simulink subsystem "Controller_v2"  (R2025b)
settings: Solver=VariableStepAuto  StartTime=0.0  StopTime=10.0  RelTol=1e-3
libraries: slpidlib x12
(part 2 of 2)

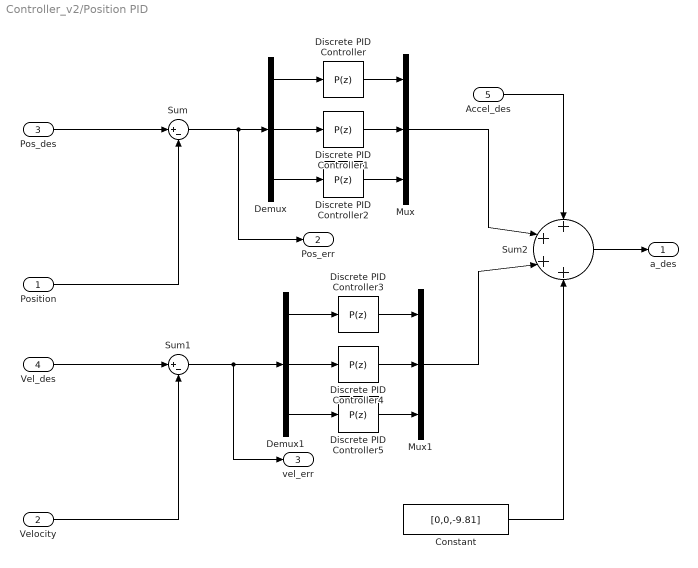
== system Controller_v2/Position PID ==
  Position : Inport
  Velocity : Inport  Port=2
  Pos_des : Inport  Port=3
  Vel_des : Inport  Port=4
  Accel_des : Inport  Port=5
  Constant : Constant  Value=[0,0,-9.81]
  Demux : Demux  Outputs=3
  Demux1 : Demux  Outputs=3
  Discrete PID Controller : slpidlib/PID Controller  Controller=P  Form=Parallel  TimeDomain=Discrete-time  UseExternalTs=off  SampleTime=1/120  IntegratorMethod=Forward Euler  FilterMethod=Forward Euler  ControllerParametersSource=internal  P=0.3  I=0  UseKiTs=off  D=0  UseExternalDerivativeSource=off  N=100  UseFilter=on  TunerSelectOption=Transfer Function Based (PID Tuner App)  InitialConditionSource=internal  InitialConditionForIntegrator=0  InitialConditionForFilter=0  DifferentiatorICPrevScaledInput=0  ExternalReset=none  TrackingMode=off  Kt=1  LimitOutput=off  SatLimitsSource=internal  UpperSaturationLimit=inf  LowerSaturationLimit=-inf  LinearizeAsGain=off  AntiWindupMode=none  Kb=1  LimitIntegrator=off  UpperIntegratorSaturationLimit=inf  LowerIntegratorSaturationLimit=-inf  POutMin=[]  POutMax=[]  IOutMin=[]  IOutMax=[]  DOutMin=[]  DOutMax=[]  NOutMin=[]  NOutMax=[]  SumOutMin=[]  SumOutMax=[]  SaturationOutMin=[]  SaturationOutMax=[]  PParamMin=[]  PParamMax=[]  IParamMin=[]  IParamMax=[]  DParamMin=[]  DParamMax=[]  NParamMin=[]  NParamMax=[]  KbParamMin=[]  KbParamMax=[]  KtParamMin=[]  KtParamMax=[]  KbOutMin=[]  KbOutMax=[]  KtOutMin=[]  KtOutMax=[]  IntegratorOutMin=[]  IntegratorOutMax=[]  FilterOutMin=[]  FilterOutMax=[]  SumI1OutMin=[]  SumI1OutMax=[]  SumI2OutMin=[]  SumI2OutMax=[]  SumI3OutMin=[]  SumI3OutMax=[]  SumI4OutMin=[]  SumI4OutMax=[]  SumDOutMin=[]  SumDOutMax=[]  DifferentiatorOutMin=[]  DifferentiatorOutMax=[]  FilterDiffOutCoefMin=[]  FilterDiffOutCoefMax=[]  ReciprocalOutMin=[]  ReciprocalOutMax=[]  SumDenOutMin=[]  SumDenOutMax=[]  SumNumOutMin=[]  SumNumOutMax=[]  DivideOutMin=[]  DivideOutMax=[]  UdiffTsProdOutMin=[]  UdiffTsProdOutMax=[]  NTsProdOutMin=[]  NTsProdOutMax=[]  UintegralTsProdOutMin=[]  UintegralTsProdOutMax=[]  UngainTsProdOutMin=[]  UngainTsProdOutMax=[]  ClampingZeroOutDataTypeStr=Inherit: Inherit via back propagation  ClampingZeroOutMin=[]  ClampingZeroOutMax=[]  FilterDenConstantOutDataTypeStr=Inherit: Inherit via back propagation  FilterDenConstantOutMin=[]  FilterDenConstantOutMax=[]  PCopyOutDataTypeStr=Inherit: Inherit via back propagation  PCopyOutMin=[]  PCopyOutMax=[]  NCopyOutDataTypeStr=Inherit: Inherit via back propagation  NCopyOutMin=[]  NCopyOutMax=[]  IntegratorContinuousStateAttributes=''  IntegratorStateMustResolveToSignalObject=off  IntegratorRTWStateStorageClass=Auto  FilterContinuousStateAttributes=''  FilterStateMustResolveToSignalObject=off  FilterRTWStateStorageClass=Auto  ParallelPVariant=InternalParameters  IdealPVariant=Disabled  IVariant=Disabled  DVariant=Disabled  IntegratorVariant=Disabled  SatVariant=Disabled  AWVariant=Disabled  PCopyVariant=Disabled  TRVariant=Disabled  FdbkBlocksVariant=Forward  IdealPFdbkVariant=Disabled  SatFdbkVariant=Disabled  DerivativeFilterVariant=Disabled  NVariant=Disabled  NCopyVariant=Disabled_SignalSpec  FilterICVariant=Disabled  IntegratorICVariant=Disabled  ExternalResetVariant=Disabled  TRSumVariant=Passthrough  SumFdbkVariant=Disabled  SumVariant=Passthrough_P  TsampFilterVariant=InternalTs  TsampNgainVariant=Passthrough  TsampIntegralVariant=Disabled_SignalSpec  ExternalSaturationOutDataTypeStr=Inherit: Same as second input  DerivativeSourceVariant=Disabled  PreIntVariant=InternalPreInt
      settings: LibrarySourceBlock=simulink/Discrete/Discrete PID Controller
  Discrete PID Controller1 : slpidlib/PID Controller  Controller=P  Form=Parallel  TimeDomain=Discrete-time  UseExternalTs=off  SampleTime=1/120  IntegratorMethod=Forward Euler  FilterMethod=Forward Euler  ControllerParametersSource=internal  P=0.3  I=0  UseKiTs=off  D=0  UseExternalDerivativeSource=off  N=100  UseFilter=on  TunerSelectOption=Transfer Function Based (PID Tuner App)  InitialConditionSource=internal  InitialConditionForIntegrator=0  InitialConditionForFilter=0  DifferentiatorICPrevScaledInput=0  ExternalReset=none  TrackingMode=off  Kt=1  LimitOutput=off  SatLimitsSource=internal  UpperSaturationLimit=inf  LowerSaturationLimit=-inf  LinearizeAsGain=off  AntiWindupMode=none  Kb=1  LimitIntegrator=off  UpperIntegratorSaturationLimit=inf  LowerIntegratorSaturationLimit=-inf  POutMin=[]  POutMax=[]  IOutMin=[]  IOutMax=[]  DOutMin=[]  DOutMax=[]  NOutMin=[]  NOutMax=[]  SumOutMin=[]  SumOutMax=[]  SaturationOutMin=[]  SaturationOutMax=[]  PParamMin=[]  PParamMax=[]  IParamMin=[]  IParamMax=[]  DParamMin=[]  DParamMax=[]  NParamMin=[]  NParamMax=[]  KbParamMin=[]  KbParamMax=[]  KtParamMin=[]  KtParamMax=[]  KbOutMin=[]  KbOutMax=[]  KtOutMin=[]  KtOutMax=[]  IntegratorOutMin=[]  IntegratorOutMax=[]  FilterOutMin=[]  FilterOutMax=[]  SumI1OutMin=[]  SumI1OutMax=[]  SumI2OutMin=[]  SumI2OutMax=[]  SumI3OutMin=[]  SumI3OutMax=[]  SumI4OutMin=[]  SumI4OutMax=[]  SumDOutMin=[]  SumDOutMax=[]  DifferentiatorOutMin=[]  DifferentiatorOutMax=[]  FilterDiffOutCoefMin=[]  FilterDiffOutCoefMax=[]  ReciprocalOutMin=[]  ReciprocalOutMax=[]  SumDenOutMin=[]  SumDenOutMax=[]  SumNumOutMin=[]  SumNumOutMax=[]  DivideOutMin=[]  DivideOutMax=[]  UdiffTsProdOutMin=[]  UdiffTsProdOutMax=[]  NTsProdOutMin=[]  NTsProdOutMax=[]  UintegralTsProdOutMin=[]  UintegralTsProdOutMax=[]  UngainTsProdOutMin=[]  UngainTsProdOutMax=[]  ClampingZeroOutDataTypeStr=Inherit: Inherit via back propagation  ClampingZeroOutMin=[]  ClampingZeroOutMax=[]  FilterDenConstantOutDataTypeStr=Inherit: Inherit via back propagation  FilterDenConstantOutMin=[]  FilterDenConstantOutMax=[]  PCopyOutDataTypeStr=Inherit: Inherit via back propagation  PCopyOutMin=[]  PCopyOutMax=[]  NCopyOutDataTypeStr=Inherit: Inherit via back propagation  NCopyOutMin=[]  NCopyOutMax=[]  IntegratorContinuousStateAttributes=''  IntegratorStateMustResolveToSignalObject=off  IntegratorRTWStateStorageClass=Auto  FilterContinuousStateAttributes=''  FilterStateMustResolveToSignalObject=off  FilterRTWStateStorageClass=Auto  ParallelPVariant=InternalParameters  IdealPVariant=Disabled  IVariant=Disabled  DVariant=Disabled  IntegratorVariant=Disabled  SatVariant=Disabled  AWVariant=Disabled  PCopyVariant=Disabled  TRVariant=Disabled  FdbkBlocksVariant=Forward  IdealPFdbkVariant=Disabled  SatFdbkVariant=Disabled  DerivativeFilterVariant=Disabled  NVariant=Disabled  NCopyVariant=Disabled_SignalSpec  FilterICVariant=Disabled  IntegratorICVariant=Disabled  ExternalResetVariant=Disabled  TRSumVariant=Passthrough  SumFdbkVariant=Disabled  SumVariant=Passthrough_P  TsampFilterVariant=InternalTs  TsampNgainVariant=Passthrough  TsampIntegralVariant=Disabled_SignalSpec  ExternalSaturationOutDataTypeStr=Inherit: Same as second input  DerivativeSourceVariant=Disabled  PreIntVariant=InternalPreInt
      settings: LibrarySourceBlock=simulink/Discrete/Discrete PID Controller
  Discrete PID Controller2 : slpidlib/PID Controller  Controller=P  Form=Parallel  TimeDomain=Discrete-time  UseExternalTs=off  SampleTime=1/120  IntegratorMethod=Forward Euler  FilterMethod=Forward Euler  ControllerParametersSource=internal  P=2.5  I=0  UseKiTs=off  D=0  UseExternalDerivativeSource=off  N=100  UseFilter=on  TunerSelectOption=Transfer Function Based (PID Tuner App)  InitialConditionSource=internal  InitialConditionForIntegrator=0  InitialConditionForFilter=0  DifferentiatorICPrevScaledInput=0  ExternalReset=none  TrackingMode=off  Kt=1  LimitOutput=off  SatLimitsSource=internal  UpperSaturationLimit=inf  LowerSaturationLimit=-inf  LinearizeAsGain=off  AntiWindupMode=none  Kb=1  LimitIntegrator=off  UpperIntegratorSaturationLimit=inf  LowerIntegratorSaturationLimit=-inf  POutMin=[]  POutMax=[]  IOutMin=[]  IOutMax=[]  DOutMin=[]  DOutMax=[]  NOutMin=[]  NOutMax=[]  SumOutMin=[]  SumOutMax=[]  SaturationOutMin=[]  SaturationOutMax=[]  PParamMin=[]  PParamMax=[]  IParamMin=[]  IParamMax=[]  DParamMin=[]  DParamMax=[]  NParamMin=[]  NParamMax=[]  KbParamMin=[]  KbParamMax=[]  KtParamMin=[]  KtParamMax=[]  KbOutMin=[]  KbOutMax=[]  KtOutMin=[]  KtOutMax=[]  IntegratorOutMin=[]  IntegratorOutMax=[]  FilterOutMin=[]  FilterOutMax=[]  SumI1OutMin=[]  SumI1OutMax=[]  SumI2OutMin=[]  SumI2OutMax=[]  SumI3OutMin=[]  SumI3OutMax=[]  SumI4OutMin=[]  SumI4OutMax=[]  SumDOutMin=[]  SumDOutMax=[]  DifferentiatorOutMin=[]  DifferentiatorOutMax=[]  FilterDiffOutCoefMin=[]  FilterDiffOutCoefMax=[]  ReciprocalOutMin=[]  ReciprocalOutMax=[]  SumDenOutMin=[]  SumDenOutMax=[]  SumNumOutMin=[]  SumNumOutMax=[]  DivideOutMin=[]  DivideOutMax=[]  UdiffTsProdOutMin=[]  UdiffTsProdOutMax=[]  NTsProdOutMin=[]  NTsProdOutMax=[]  UintegralTsProdOutMin=[]  UintegralTsProdOutMax=[]  UngainTsProdOutMin=[]  UngainTsProdOutMax=[]  ClampingZeroOutDataTypeStr=Inherit: Inherit via back propagation  ClampingZeroOutMin=[]  ClampingZeroOutMax=[]  FilterDenConstantOutDataTypeStr=Inherit: Inherit via back propagation  FilterDenConstantOutMin=[]  FilterDenConstantOutMax=[]  PCopyOutDataTypeStr=Inherit: Inherit via back propagation  PCopyOutMin=[]  PCopyOutMax=[]  NCopyOutDataTypeStr=Inherit: Inherit via back propagation  NCopyOutMin=[]  NCopyOutMax=[]  IntegratorContinuousStateAttributes=''  IntegratorStateMustResolveToSignalObject=off  IntegratorRTWStateStorageClass=Auto  FilterContinuousStateAttributes=''  FilterStateMustResolveToSignalObject=off  FilterRTWStateStorageClass=Auto  ParallelPVariant=InternalParameters  IdealPVariant=Disabled  IVariant=Disabled  DVariant=Disabled  IntegratorVariant=Disabled  SatVariant=Disabled  AWVariant=Disabled  PCopyVariant=Disabled  TRVariant=Disabled  FdbkBlocksVariant=Forward  IdealPFdbkVariant=Disabled  SatFdbkVariant=Disabled  DerivativeFilterVariant=Disabled  NVariant=Disabled  NCopyVariant=Disabled_SignalSpec  FilterICVariant=Disabled  IntegratorICVariant=Disabled  ExternalResetVariant=Disabled  TRSumVariant=Passthrough  SumFdbkVariant=Disabled  SumVariant=Passthrough_P  TsampFilterVariant=InternalTs  TsampNgainVariant=Passthrough  TsampIntegralVariant=Disabled_SignalSpec  ExternalSaturationOutDataTypeStr=Inherit: Same as second input  DerivativeSourceVariant=Disabled  PreIntVariant=InternalPreInt
      settings: LibrarySourceBlock=simulink/Discrete/Discrete PID Controller
  Discrete PID Controller3 : slpidlib/PID Controller  Controller=P  Form=Parallel  TimeDomain=Discrete-time  UseExternalTs=off  SampleTime=1/120  IntegratorMethod=Forward Euler  FilterMethod=Forward Euler  ControllerParametersSource=internal  P=2  I=1  UseKiTs=off  D=0  UseExternalDerivativeSource=off  N=100  UseFilter=on  TunerSelectOption=Transfer Function Based (PID Tuner App)  InitialConditionSource=internal  InitialConditionForIntegrator=0  InitialConditionForFilter=0  DifferentiatorICPrevScaledInput=0  ExternalReset=none  TrackingMode=off  Kt=1  LimitOutput=off  SatLimitsSource=internal  UpperSaturationLimit=inf  LowerSaturationLimit=-inf  LinearizeAsGain=off  AntiWindupMode=none  Kb=1  LimitIntegrator=off  UpperIntegratorSaturationLimit=inf  LowerIntegratorSaturationLimit=-inf  POutMin=[]  POutMax=[]  IOutMin=[]  IOutMax=[]  DOutMin=[]  DOutMax=[]  NOutMin=[]  NOutMax=[]  SumOutMin=[]  SumOutMax=[]  SaturationOutMin=[]  SaturationOutMax=[]  PParamMin=[]  PParamMax=[]  IParamMin=[]  IParamMax=[]  DParamMin=[]  DParamMax=[]  NParamMin=[]  NParamMax=[]  KbParamMin=[]  KbParamMax=[]  KtParamMin=[]  KtParamMax=[]  KbOutMin=[]  KbOutMax=[]  KtOutMin=[]  KtOutMax=[]  IntegratorOutMin=[]  IntegratorOutMax=[]  FilterOutMin=[]  FilterOutMax=[]  SumI1OutMin=[]  SumI1OutMax=[]  SumI2OutMin=[]  SumI2OutMax=[]  SumI3OutMin=[]  SumI3OutMax=[]  SumI4OutMin=[]  SumI4OutMax=[]  SumDOutMin=[]  SumDOutMax=[]  DifferentiatorOutMin=[]  DifferentiatorOutMax=[]  FilterDiffOutCoefMin=[]  FilterDiffOutCoefMax=[]  ReciprocalOutMin=[]  ReciprocalOutMax=[]  SumDenOutMin=[]  SumDenOutMax=[]  SumNumOutMin=[]  SumNumOutMax=[]  DivideOutMin=[]  DivideOutMax=[]  UdiffTsProdOutMin=[]  UdiffTsProdOutMax=[]  NTsProdOutMin=[]  NTsProdOutMax=[]  UintegralTsProdOutMin=[]  UintegralTsProdOutMax=[]  UngainTsProdOutMin=[]  UngainTsProdOutMax=[]  ClampingZeroOutDataTypeStr=Inherit: Inherit via back propagation  ClampingZeroOutMin=[]  ClampingZeroOutMax=[]  FilterDenConstantOutDataTypeStr=Inherit: Inherit via back propagation  FilterDenConstantOutMin=[]  FilterDenConstantOutMax=[]  PCopyOutDataTypeStr=Inherit: Inherit via back propagation  PCopyOutMin=[]  PCopyOutMax=[]  NCopyOutDataTypeStr=Inherit: Inherit via back propagation  NCopyOutMin=[]  NCopyOutMax=[]  IntegratorContinuousStateAttributes=''  IntegratorStateMustResolveToSignalObject=off  IntegratorRTWStateStorageClass=Auto  FilterContinuousStateAttributes=''  FilterStateMustResolveToSignalObject=off  FilterRTWStateStorageClass=Auto  ParallelPVariant=InternalParameters  IdealPVariant=Disabled  IVariant=Disabled  DVariant=Disabled  IntegratorVariant=Disabled  SatVariant=Disabled  AWVariant=Disabled  PCopyVariant=Disabled  TRVariant=Disabled  FdbkBlocksVariant=Forward  IdealPFdbkVariant=Disabled  SatFdbkVariant=Disabled  DerivativeFilterVariant=Disabled  NVariant=Disabled  NCopyVariant=Disabled_SignalSpec  FilterICVariant=Disabled  IntegratorICVariant=Disabled  ExternalResetVariant=Disabled  TRSumVariant=Passthrough  SumFdbkVariant=Disabled  SumVariant=Passthrough_P  TsampFilterVariant=InternalTs  TsampNgainVariant=Passthrough  TsampIntegralVariant=Disabled_SignalSpec  ExternalSaturationOutDataTypeStr=Inherit: Same as second input  DerivativeSourceVariant=Disabled  PreIntVariant=InternalPreInt
      settings: LibrarySourceBlock=simulink/Discrete/Discrete PID Controller
  Discrete PID Controller4 : slpidlib/PID Controller  Controller=P  Form=Parallel  TimeDomain=Discrete-time  UseExternalTs=off  SampleTime=1/120  IntegratorMethod=Forward Euler  FilterMethod=Forward Euler  ControllerParametersSource=internal  P=2  I=1  UseKiTs=off  D=0  UseExternalDerivativeSource=off  N=100  UseFilter=on  TunerSelectOption=Transfer Function Based (PID Tuner App)  InitialConditionSource=internal  InitialConditionForIntegrator=0  InitialConditionForFilter=0  DifferentiatorICPrevScaledInput=0  ExternalReset=none  TrackingMode=off  Kt=1  LimitOutput=off  SatLimitsSource=internal  UpperSaturationLimit=inf  LowerSaturationLimit=-inf  LinearizeAsGain=off  AntiWindupMode=none  Kb=1  LimitIntegrator=off  UpperIntegratorSaturationLimit=inf  LowerIntegratorSaturationLimit=-inf  POutMin=[]  POutMax=[]  IOutMin=[]  IOutMax=[]  DOutMin=[]  DOutMax=[]  NOutMin=[]  NOutMax=[]  SumOutMin=[]  SumOutMax=[]  SaturationOutMin=[]  SaturationOutMax=[]  PParamMin=[]  PParamMax=[]  IParamMin=[]  IParamMax=[]  DParamMin=[]  DParamMax=[]  NParamMin=[]  NParamMax=[]  KbParamMin=[]  KbParamMax=[]  KtParamMin=[]  KtParamMax=[]  KbOutMin=[]  KbOutMax=[]  KtOutMin=[]  KtOutMax=[]  IntegratorOutMin=[]  IntegratorOutMax=[]  FilterOutMin=[]  FilterOutMax=[]  SumI1OutMin=[]  SumI1OutMax=[]  SumI2OutMin=[]  SumI2OutMax=[]  SumI3OutMin=[]  SumI3OutMax=[]  SumI4OutMin=[]  SumI4OutMax=[]  SumDOutMin=[]  SumDOutMax=[]  DifferentiatorOutMin=[]  DifferentiatorOutMax=[]  FilterDiffOutCoefMin=[]  FilterDiffOutCoefMax=[]  ReciprocalOutMin=[]  ReciprocalOutMax=[]  SumDenOutMin=[]  SumDenOutMax=[]  SumNumOutMin=[]  SumNumOutMax=[]  DivideOutMin=[]  DivideOutMax=[]  UdiffTsProdOutMin=[]  UdiffTsProdOutMax=[]  NTsProdOutMin=[]  NTsProdOutMax=[]  UintegralTsProdOutMin=[]  UintegralTsProdOutMax=[]  UngainTsProdOutMin=[]  UngainTsProdOutMax=[]  ClampingZeroOutDataTypeStr=Inherit: Inherit via back propagation  ClampingZeroOutMin=[]  ClampingZeroOutMax=[]  FilterDenConstantOutDataTypeStr=Inherit: Inherit via back propagation  FilterDenConstantOutMin=[]  FilterDenConstantOutMax=[]  PCopyOutDataTypeStr=Inherit: Inherit via back propagation  PCopyOutMin=[]  PCopyOutMax=[]  NCopyOutDataTypeStr=Inherit: Inherit via back propagation  NCopyOutMin=[]  NCopyOutMax=[]  IntegratorContinuousStateAttributes=''  IntegratorStateMustResolveToSignalObject=off  IntegratorRTWStateStorageClass=Auto  FilterContinuousStateAttributes=''  FilterStateMustResolveToSignalObject=off  FilterRTWStateStorageClass=Auto  ParallelPVariant=InternalParameters  IdealPVariant=Disabled  IVariant=Disabled  DVariant=Disabled  IntegratorVariant=Disabled  SatVariant=Disabled  AWVariant=Disabled  PCopyVariant=Disabled  TRVariant=Disabled  FdbkBlocksVariant=Forward  IdealPFdbkVariant=Disabled  SatFdbkVariant=Disabled  DerivativeFilterVariant=Disabled  NVariant=Disabled  NCopyVariant=Disabled_SignalSpec  FilterICVariant=Disabled  IntegratorICVariant=Disabled  ExternalResetVariant=Disabled  TRSumVariant=Passthrough  SumFdbkVariant=Disabled  SumVariant=Passthrough_P  TsampFilterVariant=InternalTs  TsampNgainVariant=Passthrough  TsampIntegralVariant=Disabled_SignalSpec  ExternalSaturationOutDataTypeStr=Inherit: Same as second input  DerivativeSourceVariant=Disabled  PreIntVariant=InternalPreInt
      settings: LibrarySourceBlock=simulink/Discrete/Discrete PID Controller
  Discrete PID Controller5 : slpidlib/PID Controller  Controller=P  Form=Parallel  TimeDomain=Discrete-time  UseExternalTs=off  SampleTime=1/120  IntegratorMethod=Forward Euler  FilterMethod=Forward Euler  ControllerParametersSource=internal  P=3.5  I=1  UseKiTs=off  D=0  UseExternalDerivativeSource=off  N=100  UseFilter=on  TunerSelectOption=Transfer Function Based (PID Tuner App)  InitialConditionSource=internal  InitialConditionForIntegrator=0  InitialConditionForFilter=0  DifferentiatorICPrevScaledInput=0  ExternalReset=none  TrackingMode=off  Kt=1  LimitOutput=off  SatLimitsSource=internal  UpperSaturationLimit=inf  LowerSaturationLimit=-inf  LinearizeAsGain=off  AntiWindupMode=none  Kb=1  LimitIntegrator=off  UpperIntegratorSaturationLimit=inf  LowerIntegratorSaturationLimit=-inf  POutMin=[]  POutMax=[]  IOutMin=[]  IOutMax=[]  DOutMin=[]  DOutMax=[]  NOutMin=[]  NOutMax=[]  SumOutMin=[]  SumOutMax=[]  SaturationOutMin=[]  SaturationOutMax=[]  PParamMin=[]  PParamMax=[]  IParamMin=[]  IParamMax=[]  DParamMin=[]  DParamMax=[]  NParamMin=[]  NParamMax=[]  KbParamMin=[]  KbParamMax=[]  KtParamMin=[]  KtParamMax=[]  KbOutMin=[]  KbOutMax=[]  KtOutMin=[]  KtOutMax=[]  IntegratorOutMin=[]  IntegratorOutMax=[]  FilterOutMin=[]  FilterOutMax=[]  SumI1OutMin=[]  SumI1OutMax=[]  SumI2OutMin=[]  SumI2OutMax=[]  SumI3OutMin=[]  SumI3OutMax=[]  SumI4OutMin=[]  SumI4OutMax=[]  SumDOutMin=[]  SumDOutMax=[]  DifferentiatorOutMin=[]  DifferentiatorOutMax=[]  FilterDiffOutCoefMin=[]  FilterDiffOutCoefMax=[]  ReciprocalOutMin=[]  ReciprocalOutMax=[]  SumDenOutMin=[]  SumDenOutMax=[]  SumNumOutMin=[]  SumNumOutMax=[]  DivideOutMin=[]  DivideOutMax=[]  UdiffTsProdOutMin=[]  UdiffTsProdOutMax=[]  NTsProdOutMin=[]  NTsProdOutMax=[]  UintegralTsProdOutMin=[]  UintegralTsProdOutMax=[]  UngainTsProdOutMin=[]  UngainTsProdOutMax=[]  ClampingZeroOutDataTypeStr=Inherit: Inherit via back propagation  ClampingZeroOutMin=[]  ClampingZeroOutMax=[]  FilterDenConstantOutDataTypeStr=Inherit: Inherit via back propagation  FilterDenConstantOutMin=[]  FilterDenConstantOutMax=[]  PCopyOutDataTypeStr=Inherit: Inherit via back propagation  PCopyOutMin=[]  PCopyOutMax=[]  NCopyOutDataTypeStr=Inherit: Inherit via back propagation  NCopyOutMin=[]  NCopyOutMax=[]  IntegratorContinuousStateAttributes=''  IntegratorStateMustResolveToSignalObject=off  IntegratorRTWStateStorageClass=Auto  FilterContinuousStateAttributes=''  FilterStateMustResolveToSignalObject=off  FilterRTWStateStorageClass=Auto  ParallelPVariant=InternalParameters  IdealPVariant=Disabled  IVariant=Disabled  DVariant=Disabled  IntegratorVariant=Disabled  SatVariant=Disabled  AWVariant=Disabled  PCopyVariant=Disabled  TRVariant=Disabled  FdbkBlocksVariant=Forward  IdealPFdbkVariant=Disabled  SatFdbkVariant=Disabled  DerivativeFilterVariant=Disabled  NVariant=Disabled  NCopyVariant=Disabled_SignalSpec  FilterICVariant=Disabled  IntegratorICVariant=Disabled  ExternalResetVariant=Disabled  TRSumVariant=Passthrough  SumFdbkVariant=Disabled  SumVariant=Passthrough_P  TsampFilterVariant=InternalTs  TsampNgainVariant=Passthrough  TsampIntegralVariant=Disabled_SignalSpec  ExternalSaturationOutDataTypeStr=Inherit: Same as second input  DerivativeSourceVariant=Disabled  PreIntVariant=InternalPreInt
      settings: LibrarySourceBlock=simulink/Discrete/Discrete PID Controller
  Mux : Mux  Inputs=3
  Mux1 : Mux  Inputs=3
  Sum : Sum  Inputs=|+-
  Sum1 : Sum  Inputs=|+-
  Sum2 : Sum  Inputs=++++
  a_des : Outport
  Pos_err : Outport  Port=2
  vel_err : Outport  Port=3
  wires:
  Mux1/1 -> Sum2/3
  Demux1/3 -> Discrete PID Controller5/1
  Demux1/2 -> Discrete PID Controller4/1
  Discrete PID Controller5/1 -> Mux1/3
  Discrete PID Controller3/1 -> Mux1/1
  Demux1/1 -> Discrete PID Controller3/1
  Discrete PID Controller4/1 -> Mux1/2
  Mux/1 -> Sum2/2
  Discrete PID Controller2/1 -> Mux/3
  Discrete PID Controller1/1 -> Mux/2
  Discrete PID Controller/1 -> Mux/1
  Demux/3 -> Discrete PID Controller2/1
  Demux/2 -> Discrete PID Controller1/1
  Demux/1 -> Discrete PID Controller/1
  Sum2/1 -> a_des/1
  Constant/1 -> Sum2/4
  Accel_des/1 -> Sum2/1
  Sum/1 -> Pos_err/1, Demux/1
  Sum1/1 -> vel_err/1, Demux1/1
  Velocity/1 -> Sum1/2
  Vel_des/1 -> Sum1/1
  Position/1 -> Sum/2
  Pos_des/1 -> Sum/1

== matlab function Controller_v2/MATLAB Function ==
  data: pitch_deg input; T_top_N output; yaw_deg input; top_pre_percent input; bottom_pre_percent input; max_total_thrust input; T_bottom_N output; y_gimbal_rad output; z_gimbal_rad output
function [T_top_N, T_bottom_N, ...
          y_gimbal_rad, z_gimbal_rad] = ...
    controller_to_physics( ...
        pitch_deg, yaw_deg, ...
        top_pre_percent, bottom_pre_percent, ...
        max_total_thrust)
%CONTROLLER_TO_PHYSICS Convert controller signals to physics inputs.
%
% Inputs:
%   pitch_deg           Pitch-gimbal command in degrees
%   yaw_deg             Yaw-gimbal command in degrees
%   top_pre_percent     Top command after roll mix and saturation,
%                       but before the 0.72 exponent
%   bottom_pre_percent  Bottom command after roll mix and saturation,
%                       but before the 0.72 exponent
%   max_total_thrust    Combined maximum thrust, currently 28 N
%
% Outputs:
%   T_top_N             Top-propeller thrust in newtons
%   T_bottom_N          Bottom-propeller thrust in newtons
%   y_gimbal_rad        Pitch command in radians
%   z_gimbal_rad        Yaw command in radians

% Defensive command saturation
top_pre_percent = min(max(top_pre_percent, 0), 100);
bottom_pre_percent = min(max(bottom_pre_percent, 0), 100);

max_total_thrust = max(max_total_thrust, 0);
max_each_thrust = max_total_thrust / 2;

% Pre-exponent percentages represent normalized physical thrust
T_top_N = max_each_thrust * top_pre_percent / 100;
T_bottom_N = max_each_thrust * bottom_pre_percent / 100;

% Controller outputs degrees; physics model expects radians
y_gimbal_rad = pitch_deg * pi / 180;
z_gimbal_rad = yaw_deg * pi / 180;

end

== matlab function Controller_v2/Thrust Direction Error ==
  data: q_body_to_ned input; thrust_dir_world output; thrust_dir_world_des input; dir_error_world output; dir_error_body output; thrust_dir_body_des output
function [thrust_dir_world, dir_error_world, ...
          dir_error_body, thrust_dir_body_des] = ...
    thrust_direction_error(q_body_to_ned, thrust_dir_world_des)
%#codegen

% Normalise quaternion
q_norm = norm(q_body_to_ned);

if q_norm < 1e-9
    q = [1.0; 0.0; 0.0; 0.0];
else
    q = q_body_to_ned / q_norm;
end

% Body +X is the physical thrust axis
thrust_axis_body = [1.0; 0.0; 0.0];

% Transform body +X into NED
thrust_dir_world = body2ned(thrust_axis_body, q);
thrust_dir_world = thrust_dir_world / norm(thrust_dir_world);

% Normalise desired world direction
if norm(thrust_dir_world_des) < 1e-6
    desired_world = [0.0; 0.0; -1.0];
else
    desired_world = ...
        thrust_dir_world_des / norm(thrust_dir_world_des);
end

% Error rotation axis, expressed in NED
dir_error_world = cross(thrust_dir_world, desired_world);

% Express error in body coordinates
dir_error_body = ned2body(dir_error_world, q);

% Desired thrust direction expressed in body coordinates
thrust_dir_body_des = ned2body(desired_world, q);

end

== matlab function Controller_v2/Tilt Compensated Thrust ==
  data: F_outer input; Fx_cmd output; thrust_dir_ned_des input; q_body_to_ned input; max_thrust input; minimum_tilt_cosine input; cos_tilt output; upward_force_target output; body_x_axis_ned output
function [Fx_cmd, cos_tilt, upward_force_target, ...
          body_x_axis_ned] = ...
    tilt_compensated_thrust( ...
        F_outer, thrust_dir_ned_des, q_body_to_ned, ...
        max_thrust, minimum_tilt_cosine)
%#codegen

%% Normalize quaternion

q_norm = norm(q_body_to_ned);

if q_norm < 1e-9
    q = [1.0;0.0;0.0;0.0];
else
    q = q_body_to_ned / q_norm;
end

%% Normalize desired thrust direction

if norm(thrust_dir_ned_des) < 1e-6
    desired_direction_ned = [0.0;0.0;-1.0];
else
    desired_direction_ned = ...
        thrust_dir_ned_des / norm(thrust_dir_ned_des);
end

%% Current body +X direction in NED

body_x_axis_ned = body2ned([1.0;0.0;0.0],q);
body_x_axis_ned = body_x_axis_ned / norm(body_x_axis_ned);

%% Current tilt relative to NED Up

ned_up = [0.0;0.0;-1.0];

cos_tilt_raw = dot(body_x_axis_ned,ned_up);

cos_tilt = min(max( ...
    cos_tilt_raw, minimum_tilt_cosine), 1.0);

%% Required upward component of desired force

upward_force_target = max( ...
    -F_outer * desired_direction_ned(3), 0.0);

%% Compensate for current vehicle tilt

Fx_cmd = upward_force_target / cos_tilt;

Fx_cmd = min(max(Fx_cmd,0.0),max_thrust);

end

== matlab function Controller_v2/Force to Thrust Command ==
  data: F_des_world_limited input; thrust_dir_world_des output; Fx_cmd_outer output; F_mag output; max_thrust input
function [thrust_dir_world_des, Fx_cmd_outer, F_mag] = ...
    force_to_thrust_command(F_des_world_limited, max_thrust)


% Magnitude of requested world-frame force
F_mag = norm(F_des_world_limited);

% Handle a nearly zero force request
if F_mag < 1e-3
    % Default world direction is upward in NED
    thrust_dir_world_des = [0.0; 0.0; -1.0];
    Fx_cmd_outer = 0.0;
else
    % Unit vector describing the desired world thrust direction
    thrust_dir_world_des = F_des_world_limited / F_mag;

    % Limit total commanded thrust to 28 N
    Fx_cmd_outer = min(max(F_mag, 0.0), max_thrust);
end

end

== matlab function Controller_v2/Position Tilt Limiter ==
  data: F_requested input; F_limited output
function F_limited = limit_position_tilt(F_requested)

F_limited = F_requested;

% NED convention: negative Down force is upward force
upward_force = max(-F_limited(3), 0.0);
F_limited(3) = -upward_force;

max_horizontal_force = upward_force * tan(20.0 * pi / 180.0);

horizontal_force = hypot(F_limited(1), F_limited(2));

if horizontal_force > max_horizontal_force
    if horizontal_force > 1e-6
        scale = max_horizontal_force / horizontal_force;

        F_limited(1) = F_limited(1) * scale;
        F_limited(2) = F_limited(2) * scale;
    else
        F_limited(1) = 0.0;
        F_limited(2) = 0.0;
    end
end

end

== matlab function Controller_v2/Roll Error Reference ==
  settings: updateMethod=DISCRETE
  data: q_body_to_ned input; roll_error output; reset_roll_reference input
function roll_error = roll_error_reference( ...
    q_body_to_ned, reset_roll_reference)
%#codegen

persistent roll_zero_x_world
persistent roll_zero_y_world
persistent reference_valid

if isempty(reference_valid)
    roll_zero_x_world = zeros(3,1);
    roll_zero_y_world = zeros(3,1);
    reference_valid = false;
end

% Normalise attitude quaternion
q_norm = norm(q_body_to_ned);

if q_norm < 1e-9
    q = [1.0; 0.0; 0.0; 0.0];
else
    q = q_body_to_ned / q_norm;
end

body_x_world = body2ned([1.0;0.0;0.0], q);
body_y_world = body2ned([0.0;1.0;0.0], q);

body_x_world = body_x_world / norm(body_x_world);
body_y_world = body_y_world / norm(body_y_world);

% Capture the initial roll reference
if reset_roll_reference || ~reference_valid
    roll_zero_x_world = body_x_world;
    roll_zero_y_world = body_y_world;
    reference_valid = true;
end

% Transport the original body-Y reference to the current thrust direction
R_zero_to_current = rotation_between_vectors( ...
    roll_zero_x_world, body_x_world);

roll_reference_y_world = ...
    R_zero_to_current * roll_zero_y_world;

% Project both Y vectors onto the plane normal to current body +X
roll_reference_y_world = roll_reference_y_world ...
    - body_x_world * dot(roll_reference_y_world, body_x_world);

current_y_world = body_y_world ...
    - body_x_world * dot(body_y_world, body_x_world);

reference_norm = norm(roll_reference_y_world);
current_norm = norm(current_y_world);

if reference_norm > 1e-6 && current_norm > 1e-6
    roll_reference_y_world = ...
        roll_reference_y_world / reference_norm;

    current_y_world = current_y_world / current_norm;

    roll_error = atan2( ...
        dot(body_x_world, ...
            cross(current_y_world, roll_reference_y_world)), ...
        dot(current_y_world, roll_reference_y_world));
else
    roll_error = 0.0;
end

end


function R = rotation_between_vectors(a, b)
% Minimal rotation matrix that aligns unit vector a with unit vector b.

a = a / norm(a);
b = b / norm(b);

cross_ab = cross(a,b);
dot_ab = max(min(dot(a,b), 1.0), -1.0);

if dot_ab > 1.0 - 1e-10
    R = eye(3);

elseif dot_ab < -1.0 + 1e-10
    % Handle the 180-degree case
    if abs(a(1)) <= abs(a(2)) && abs(a(1)) <= abs(a(3))
        candidate = [1.0;0.0;0.0];
    elseif abs(a(2)) <= abs(a(3))
        candidate = [0.0;1.0;0.0];
    else
        candidate = [0.0;0.0;1.0];
    end

    axis = cross(a,candidate);
    axis = axis / norm(axis);

    R = -eye(3) + 2.0*(axis*axis.');

else
    K = [0.0,         -cross_ab(3),  cross_ab(2);
         cross_ab(3),  0.0,         -cross_ab(1);
        -cross_ab(2),  cross_ab(1),  0.0];

    R = eye(3) + K + (K*K)/(1.0 + dot_ab);
end

end

== matlab function Controller_v2/Body Force Allocation ==
  data: Fx_cmd input; F_body output; M_cmd_body input; r_engine_body input
function F_body = body_force_allocation( ...
    Fx_cmd, M_cmd_body, r_engine_body)
%#codegen

rx = r_engine_body(1);
ry = r_engine_body(2);
rz = r_engine_body(3);

F_body = zeros(3,1);

% Required axial thrust
F_body(1) = Fx_cmd;

% Lateral body forces required to produce body-Z and body-Y moments
F_body(2) = ...
    (M_cmd_body(3) + ry*Fx_cmd) / rx;

F_body(3) = ...
    (rz*Fx_cmd - M_cmd_body(2)) / rx;

end

== matlab function Controller_v2/Body Force to Actuator Commands ==
  data: F_body input; pitch_servo_raw_deg output; max_thrust input; yaw_servo_raw_deg output; base_thrust_raw_percent output; F_body_magnitude output
function [pitch_servo_raw_deg, yaw_servo_raw_deg, ...
          base_thrust_raw_percent, F_body_magnitude] = ...
    body_force_to_actuator_commands(F_body,max_thrust)
%#codegen

Fx = F_body(1);
Fy = F_body(2);
Fz = F_body(3);

% Required gimbal angles
pitch_servo_raw_deg = atan2(Fz,Fx) * 180.0/pi;
yaw_servo_raw_deg   = atan2(Fy,Fx) * 180.0/pi;

% Total requested force magnitude
F_body_magnitude = norm(F_body);

% Convert force magnitude into percentage of maximum thrust
base_thrust_raw_percent = ...
    F_body_magnitude * 100.0/max_thrust;

end

== matlab function Controller_v2/Battery Voltage Compensation ==
  data: base_thrust_raw_percent input; base_thrust_scaled_percent output; battery_voltage input; voltage_scale output; raw_voltage_scale output; battery_fresh input; nominal_battery_voltage input; minimum_valid_battery_voltage input; voltage_scale_exponent input; minimum_voltage_scale input; maximum_voltage_scale input
function [base_thrust_scaled_percent, voltage_scale, ...
          raw_voltage_scale] = ...
    battery_voltage_compensation( ...
        base_thrust_raw_percent, ...
        battery_voltage, battery_fresh, ...
        nominal_battery_voltage, ...
        minimum_valid_battery_voltage, ...
        voltage_scale_exponent, ...
        minimum_voltage_scale, ...
        maximum_voltage_scale)
%#codegen

% Default to no compensation
raw_voltage_scale = 1.0;
voltage_scale = 1.0;

% Only trust a fresh, valid battery measurement
if battery_fresh && ...
        battery_voltage > minimum_valid_battery_voltage

    raw_voltage_scale = ...
        nominal_battery_voltage / battery_voltage;

    voltage_scale = ...
        raw_voltage_scale^voltage_scale_exponent;

    voltage_scale = min(max( ...
        voltage_scale, minimum_voltage_scale), ...
        maximum_voltage_scale);
end

% Apply voltage compensation
base_thrust_scaled_percent = ...
    base_thrust_raw_percent * voltage_scale;

% Limit final base throttle
base_thrust_scaled_percent = min(max( ...
    base_thrust_scaled_percent,0.0),100.0);

end

== matlab function Controller_v2/Roll Mix and Thrust Linearisation ==
  data: base_thrust_scaled_percent input; thrust_top_percent output; Mx_cmd_body input; thrust_bottom_percent output; roll_mix output; voltage_scale input; roll_mix_offset input; maximum_roll_mix input; thrust_exponent input; thrust_top_prelinear output; thrust_bottom_prelinear output
function [thrust_top_percent, thrust_bottom_percent, ...
          roll_mix, thrust_top_prelinear, ...
          thrust_bottom_prelinear] = ...
    roll_mix_and_linearise( ...
        base_thrust_scaled_percent, ...
        Mx_cmd_body, voltage_scale, ...
        roll_mix_offset, maximum_roll_mix, ...
        thrust_exponent)
%#codegen

%% Differential roll command

roll_mix = Mx_cmd_body * voltage_scale;

% Constant trim for the measured roll bias
roll_mix = roll_mix + roll_mix_offset;

% Limit differential throttle
roll_mix = min(max( ...
    roll_mix,-maximum_roll_mix),maximum_roll_mix);

%% Mix common and differential throttle

% Positive roll mix:
% top propeller increases, bottom propeller decreases
thrust_top_prelinear = ...
    base_thrust_scaled_percent + roll_mix;

thrust_bottom_prelinear = ...
    base_thrust_scaled_percent - roll_mix;

% Individual propeller limits
thrust_top_prelinear = min(max( ...
    thrust_top_prelinear,0.0),100.0);

thrust_bottom_prelinear = min(max( ...
    thrust_bottom_prelinear,0.0),100.0);

%% Thrust linearisation

thrust_top_percent = 100.0 * ...
    (thrust_top_prelinear/100.0)^thrust_exponent;

thrust_bottom_percent = 100.0 * ...
    (thrust_bottom_prelinear/100.0)^thrust_exponent;

end
